simulink model "q_aero2_pitch_from_yaw_step"  (R2025a)
settings: Solver=ode1  StartTime=0.0  StopTime=90  FixedStep=0.002  RelTol=1e-3  EnableMultiTasking=on
undefined symbols (not defined in the file or in its folder): HIL, qc_get_step_size
libraries: quarc_library x4
settings Model: SimulationMode=external  ExtModeTrigDuration=20001  Creator=MLevis  LastModifiedBy=khanh
settings SolverCC: AlgebraicLoopSolver=TrustRegion  PositivePriorityOrder=on
settings DataIOCC: LimitDataPoints=on  SaveFormat=Array  SignalLoggingSaveFormat=ModelDataLogs  ReturnWorkspaceOutputs=off
settings OptimizationCC: ExpressionDepthLimit=2147483647.0
settings DebuggingCC: UnderspecifiedInitializationDetection=Classic  MergeDetectMultiDrivingBlocksExec=none  SolverPrmCheckMsg=warning  FcnCallInpInsideContextMsg=warning  UnconnectedInputMsg=warning  UnconnectedOutputMsg=warning  UnconnectedLineMsg=warning  StateNameClashWarn=warning  SFUnexpectedBacktrackingDiag=warning  SFNoUnconditionalDefaultTransitionDiag=warning  SFExecutionAtInitializationDiag=none  ArithmeticOperatorsInVariantConditions=warning
settings ModelReferenceCC: EnableRefExpFcnMdlSchedulingChecks=on  PropagateSignalLabelsOutOfModel=off
settings SFSimCC: SimUseLocalCustomCode=off  CustomCodeUndefinedFunction=UseInterfaceOnly
settings RTWCC: SystemTargetFile=quarc_win64.tlc  TemplateMakefile=quarc_default_tmf  RTWUseLocalCustomCode=off  Toolchain=QUARC win64 | nmake (64-bit Windows)  BuildConfiguration=Faster Runs  GPUComputeCapability=3.5  DLArmComputeVersion=19.05  Description=QUARC Win64 Target Using Toolchain
settings CodeAppCC: StateflowObjectComments=on
settings STFCustomTargetCC: SystemTargetFile=quarc_win64.tlc  MultiwordLength=2048.0  DynamicStringBufferSize=256.0  ConcurrentExecutionCompliant=on  UseToolchainInfoCompliant=on
settings GRTTargetCC: ExtMode=on  ExtModeMexFile=quarc_comm  TargetLangStandard=C89/C90 (ANSI)  ParMdlRefBuildCompliant=off  CompOptLevelCompliant=off  CombineOutputUpdateFcns=off  MatFileLogging=off  CPPClassGenCompliant=off  GRTInterface=on
settings ConfigComp: CovMetricSettings=dw  CovSaveCumulativeToWorkspaceVar=on  CovSaveSingleToWorkspaceVar=on  CovExternalEMLEnable=off  CovSFcnEnable=off

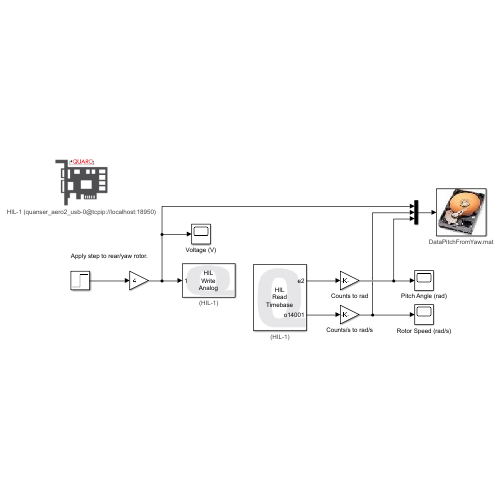
[thumbnail: Simulink's stored preview of the top-level diagram]
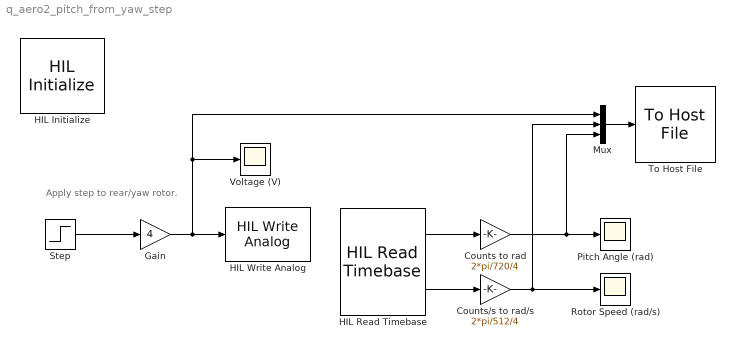
== system q_aero2_pitch_from_yaw_step ==
  note: Apply step to rear/yaw rotor.
  Counts to rad : Gain  Gain=2*pi/720/4
  Counts/s to rad/s : Gain  Gain=2*pi/512/4
  Gain : Gain  Gain=4
  HIL Initialize : quarc_library/Data Acquisition/Generic/Configuration/HIL Initialize  Priority=-99  object_name=HIL-1  board_type=quanser_aero2_usb  board_number=0@tcpip://localhost:18950  board_options=""  exclusive=off  active=off  hardware_clocks=[0]  clock_modes=[]  initial_clock_frequencies=[]  set_clock_params_at_start=off  set_clock_params_at_switch_in=off  set_clock_frequencies_at_start=off  set_clock_frequencies_at_switch_in=off  analog_input_channels=[0:1]  analog_input_configurations=[]  analog_input_maximums=3  analog_input_minimums=-3  set_analog_input_params_at_start=off  set_analog_input_params_at_switch_in=off  analog_output_channels=[0:1]  analog_output_maximums=24  analog_output_minimums=-24  initial_analog_outputs=[0]  final_analog_outputs=[0]  watchdog_analog_outputs=[0]  set_analog_output_params_at_start=off  set_analog_output_params_at_switch_in=off  set_analog_outputs_at_start=on  set_analog_outputs_at_switch_in=off  set_analog_outputs_at_terminate=on  set_analog_outputs_at_switch_out=off  set_analog_outputs_on_watchdog=on  digital_input_channels=[]  digital_output_channels=[0:1]  digital_output_configuration=[]  initial_digital_outputs=[1]  final_digital_outputs=[0]  watchdog_digital_outputs=[0]  set_digital_output_params_at_start=off  set_digital_output_params_at_switch_in=off  set_digital_outputs_at_start=on  set_digital_outputs_at_switch_in=off  set_digital_outputs_at_terminate=on  set_digital_outputs_at_switch_out=off  set_digital_outputs_on_watchdog=on  encoder_channels=[0:3]  quadrature=[4]  encoder_filter_frequency=[]  initial_encoder_counts=[0]  set_encoder_params_at_start=off  set_encoder_params_at_switch_in=off  set_encoder_counts_at_start=on  set_encoder_counts_at_switch_in=off  pwm_channels=[]  pwm_modes=[]  pwm_frequency=[]  pwm_configuration=[]  pwm_alignment=[]  pwm_polarity=[]  pwm_leading_deadband=[]  pwm_trailing_deadband=[]  initial_pwm_outputs=[]  final_pwm_outputs=[]  watchdog_pwm_outputs=[]  set_pwm_params_at_start=off  set_pwm_params_at_switch_in=off  set_pwm_outputs_at_start=off  set_pwm_outputs_at_switch_in=off  set_pwm_outputs_at_terminate=off  set_pwm_outputs_at_switch_out=off  set_pwm_outputs_on_watchdog=off  other_output_channels=[11000:11002]  initial_other_outputs=[0 1 0]  final_other_outputs=[1 0 0]  watchdog_other_outputs=[0 0 1]  set_other_outputs_at_start=on  set_other_outputs_at_switch_in=off  set_other_outputs_at_terminate=on  set_other_outputs_at_switch_out=off  set_other_outputs_on_watchdog=on
  HIL Read Timebase : quarc_library/Data Acquisition/Generic/Timebases/HIL Read Timebase  object_name=HIL-1  clock=0  analog_channels=[]  encoder_channels=[2]  digital_channels=[]  other_channels=[14001]  active=on  vector_output=off  data_type_mode=Inherit via back propagation  encoder_data_type=double  digital_data_type=boolean  overflow_mode=Error on overflow  samples_in_buffer=max(ceil(1/qc_get_step_size), 1)
  HIL Write Analog : quarc_library/Data Acquisition/Generic/Immediate I//O/HIL Write Analog  object_name=HIL-1  channels=1  sample_time=-1  active=off  vector_input=off
  Mux : Mux  Inputs=3
  Pitch Angle (rad) : Scope
      settings: ActiveDisplayYMinimum=-0.020180369476184432  ActiveDisplayYMaximum=0.18162332528565991  DataLoggingVariableName=Data_AeroModel_Pitch
  Rotor Speed (rad/s) : Scope
      settings: ActiveDisplayYMinimum=-9.9364384710788709  ActiveDisplayYMaximum=89.427946239709854  DataLoggingVariableName=Data_AeroModel_Rotor
  Step : Step  SampleTime=0
  To Host File : quarc_library/Sinks/To Host/To Host File  source=Specify via dialog (do not evaluate)  file_name=DataPitchFromYaw.mat  variable_name=PitchFromYaw  decimation=1  sample_time=-1  file_format=MAT-file v.4  options=No header or footer  append=off  final_file_name=DataPitchFromYaw.mat  encoding=Default  bitrate=2000000
  Voltage (V) : Scope
      settings: ActiveDisplayYMinimum=-0.49999999999999989  ActiveDisplayYMaximum=4.5  DataLoggingVariableName=Data_AeroModel_Vm
  wires:
  Step/1 -> Gain/1
  Counts to rad/1 -> Mux/3, Pitch Angle (rad)/1
  Counts/s to rad/s/1 -> Mux/2, Rotor Speed (rad/s)/1
  Gain/1 -> HIL Write Analog/1, Mux/1, Voltage (V)/1
  Mux/1 -> To Host File/1
  HIL Read Timebase/1 -> Counts to rad/1
  HIL Read Timebase/2 -> Counts/s to rad/s/1
